simulink model "bicycle_2dof"  (R2026b)
settings: Solver=VariableStepAuto
undefined symbols (not defined in the file): Params
settings Model: Creator=andrei  LastModifiedBy=andrei

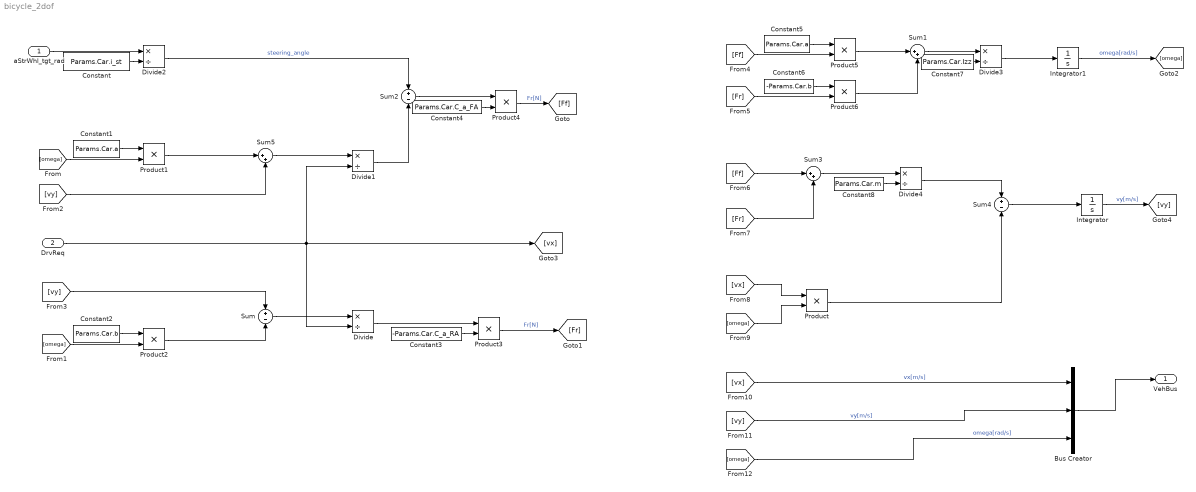
== system bicycle_2dof ==
  aStrWhl_tgt_rad : Inport
  DrvReq : Inport  Port=2
  Bus Creator : BusCreator  Inputs=3
  Constant : Constant  Value=Params.Car.i_st
  Constant1 : Constant  Value=Params.Car.a
  Constant2 : Constant  Value=Params.Car.b
  Constant3 : Constant  Value=-Params.Car.C_a_RA
  Constant4 : Constant  Value=Params.Car.C_a_FA
  Constant5 : Constant  Value=Params.Car.a
  Constant6 : Constant  Value=-Params.Car.b
  Constant7 : Constant  Value=Params.Car.Izz
  Constant8 : Constant  Value=Params.Car.m
  Divide{,1..4} (5 alike) : Product  Inputs=*/
  Integrator : Integrator
  Integrator1 : Integrator
  Product{,1..6} (7 alike) : Product
  Sum : Sum  Inputs=+-
  Sum1 : Sum  Inputs=|++
  Sum2 : Sum  Inputs=+-
  Sum3 : Sum  Inputs=|++
  Sum4 : Sum  Inputs=+-
  Sum5 : Sum  Inputs=|++
  VehBus : Outport
  wires:
  aStrWhl_tgt_rad/1 -> Divide2/1
  Divide2/1 -> Sum2/1  "steering_angle"
  [omega] -> Product1/2
  Product1/1 -> Sum5/1
  [vy] -> Sum5/2
  DrvReq/1 -> Divide/2, Divide1/2, [vx]
  Sum5/1 -> Divide1/1
  Divide1/1 -> Sum2/2
  [omega] -> Product2/2
  [vy] -> Sum/1
  Product2/1 -> Sum/2
  Sum/1 -> Divide/1
  Product5/1 -> Sum1/1
  Product6/1 -> Sum1/2
  Sum1/1 -> Divide3/1
  Divide3/1 -> Integrator1/1
  Integrator1/1 -> [omega]  "omega[rad/s]"
  [Ff] -> Sum3/1
  [Fr] -> Sum3/2
  Sum3/1 -> Divide4/1
  Divide4/1 -> Sum4/1
  [vx] -> Product/1
  [omega] -> Product/2
  Product/1 -> Sum4/2
  Sum4/1 -> Integrator/1
  Integrator/1 -> [vy]  "vy[m/s]"
  [vx] -> Bus Creator/1  "vx[m/s]"
  [vy] -> Bus Creator/2  "vy[m/s]"
  [omega] -> Bus Creator/3  "omega[rad/s]"
  Bus Creator/1 -> VehBus/1
  Constant/1 -> Divide2/2
  Constant1/1 -> Product1/1
  Constant2/1 -> Product2/1
  Sum2/1 -> Product4/1
  Product4/1 -> [Ff]  "Fr[N]"
  [Ff] -> Product5/2
  Constant5/1 -> Product5/1
  [Fr] -> Product6/2
  Constant6/1 -> Product6/1
  Constant7/1 -> Divide3/2
  Constant8/1 -> Divide4/2
  Constant4/1 -> Product4/2
  Product3/1 -> [Fr]  "Fr[N]"
  Divide/1 -> Product3/1
  Constant3/1 -> Product3/2
